simulink model "case_13_hard_brake"  (R2025b)
settings: Solver=VariableStepAuto  StartTime=0.0  StopTime=90  RelTol=1e-3
settings Model: Creator=sanborkl  LastModifiedBy=sanborkl

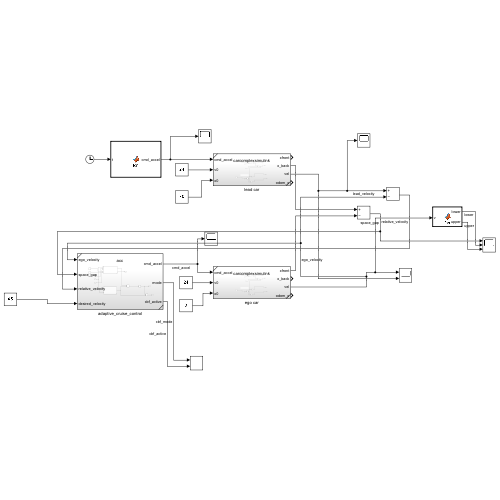
[thumbnail: Simulink's stored preview of the top-level diagram]
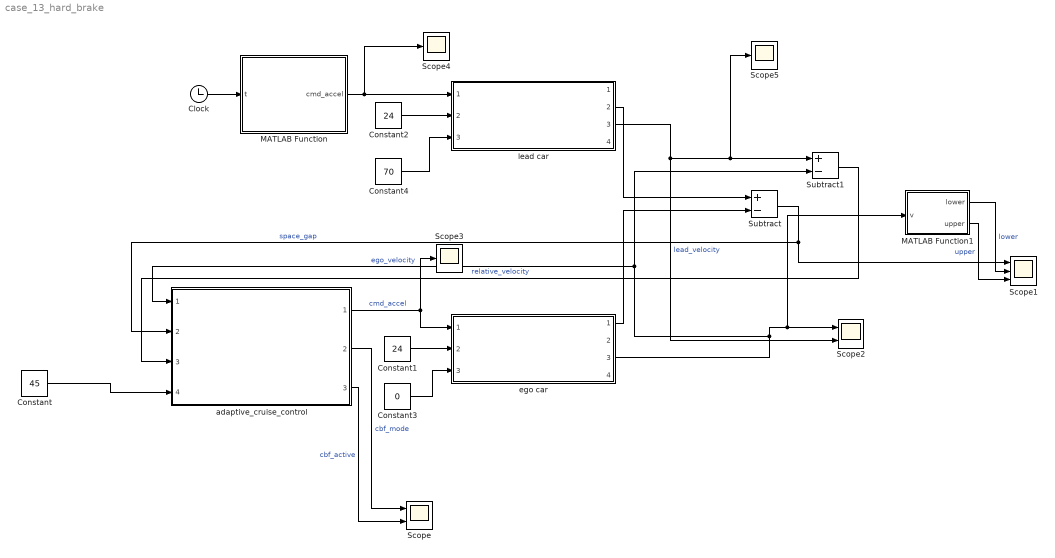
== system case_13_hard_brake ==
  Clock : Clock
  Constant : Constant  Value=45
  Constant1 : Constant  Value=24
  Constant2 : Constant  Value=24
  Constant3 : Constant  Value=0
  Constant4 : Constant  Value=70
  MATLAB Function : MATLAB Function  TreatAsAtomicUnit=on
  MATLAB Function1 : MATLAB Function  TreatAsAtomicUnit=on
  Scope : Scope  NumInputPorts=2
      settings: ActiveDisplayYMinimum=0.9  ActiveDisplayYMaximum=1.1
  Scope1 : Scope  NumInputPorts=3
      settings: ActiveDisplayYMinimum=-5.8025525665703395  ActiveDisplayYMaximum=73.711394729618917  YLabel=m
  Scope2 : Scope  NumInputPorts=2
      settings: ActiveDisplayYMinimum=-3.7568145663376993  ActiveDisplayYMaximum=33.8113310970393  YLabel=m/s  DataLoggingVariableName=ScopeData2
  Scope3 : Scope
      settings: ActiveDisplayYMinimum=-3.37975  ActiveDisplayYMaximum=0.4177499999999994  YLabel=m/s^2  DataLoggingVariableName=ScopeData3
  Scope4 : Scope
      settings: ActiveDisplayYMinimum=-5.625  ActiveDisplayYMaximum=0.62499999999999989  DataLoggingVariableName=ScopeData4
  Scope5 : Scope
      settings: ActiveDisplayYMinimum=-3.7499999999999991  ActiveDisplayYMaximum=33.75  YLabel=m/s  DataLoggingVariableName=ScopeData12
  Subtract : Sum  Inputs=+-
  Subtract1 : Sum  Inputs=+-
  adaptive_cruise_control : Subsystem  ReferencedSubsystem=acc
  ego car : Subsystem  ReferencedSubsystem=carcomplexsimulink
  lead car : Subsystem  ReferencedSubsystem=carcomplexsimulink
  wires:
  ego car/3 -> Scope2/1, MATLAB Function1/1(v), Subtract1/2, adaptive_cruise_control/1  "ego_velocity"
  adaptive_cruise_control/1 -> ego car/1, Scope3/1  "cmd_accel"
  Constant1/1 -> ego car/2
  Subtract1/1 -> adaptive_cruise_control/3  "relative_velocity"
  lead car/3 -> Scope2/2, Scope5/1, Subtract1/1  "lead_velocity"
  Constant3/1 -> ego car/3
  Constant2/1 -> lead car/2
  adaptive_cruise_control/2 -> Scope/1  "cbf_mode"
  lead car/2 -> Subtract/1
  adaptive_cruise_control/3 -> Scope/2  "cbf_active"
  Constant/1 -> adaptive_cruise_control/4
  ego car/1 -> Subtract/2
  Subtract/1 -> Scope1/1, adaptive_cruise_control/2  "space_gap"
  Constant4/1 -> lead car/3
  MATLAB Function/1(cmd_accel) -> lead car/1, Scope4/1
  Clock/1 -> MATLAB Function/1(t)
  MATLAB Function1/1(lower) -> Scope1/2  "lower"
  MATLAB Function1/2(upper) -> Scope1/3  "upper"

== matlab function case_13_hard_brake/MATLAB Function ==
  data: t input; cmd_accel output
function cmd_accel = fcn(t)

if t <= 10
    cmd_accel = 0;
else
    cmd_accel = -5;
end

== matlab function case_13_hard_brake/MATLAB Function1 ==
  data: v input; lower output; upper output
function [lower, upper] = fcn(v)

lower = 2 * v + 5;
upper = 2 * v + 15;
